simulink model "acf_force_control_simple"  (R2026b)
settings: Solver=ode4  StopTime=4  FixedStep=1.0000000000000001e-05
InitFcn:
  | acf_select_actuator(bdroot);
model workspace (MAT data in the model file):
  acfControlVersion = 'inertial-delivery-v8'
  acfImplementation = 'simple'
  acfLayoutVersion = 1
  p : object (value not decoded)
  pCompliant : object (value not decoded)
  pNearContact : object (value not decoded)
  pNoSprings : object (value not decoded)
  pRecommended : object (value not decoded)
symbols that are objects in the model workspace (value not decoded): p
undefined symbols (not defined in the file): DiscIntNeverNeededParam
(part 3 of 3)

== system acf_force_control_simple/Force controller/Coil PI and PID/Measured motion feedforward ==
  Acceleration FF audit native rate : ZeroOrderHold  SampleTime=p.sim.step
  Acceleration FF audit vector : Mux  Inputs=2
  Acceleration FF native log : ToWorkspace  VariableName=acceleration_feedforward_log  SaveFormat=Timeseries  SampleTime=-1
  Acceleration FF prediction time : Gain  Gain=p.inertial.accelerationPrediction_s
  Causal acceleration for current FF : Sum
  Filtered measured acceleration rate : DiscreteTransferFcn  Numerator=p.d.accelerationPrediction.derivativeNumerator  Denominator=p.d.accelerationPrediction.derivativeDenominator  SampleTime=p.force.sampleTime
  Geometry current feedforward : Gain  Gain=(p.contact.geometryFeedforwardScale/p.d.coilForceConstant_model_N_A)*double(p.force.feedforwardEnabled)
  Guide Coulomb friction current : Gain  Gain=(p.inertial.guideFrictionFeedforwardScale*p.coil.coulombForce/p.d.coilForceConstant_model_N_A)*double(p.force.feedforwardEnabled)
  Guide friction direction : Trigonometry  Operator=tanh
  Guide friction feedforward : Sum
  Guide friction velocity scale : Gain  Gain=1/p.coil.frictionSpeed
  Guide viscous friction current : Gain  Gain=(p.inertial.guideFrictionFeedforwardScale*p.coil.viscousFriction/p.d.coilForceConstant_model_N_A)*double(p.force.feedforwardEnabled)
  Identified guide prediction time : Gain  Gain=p.inertial.guideVelocityPrediction_s
  Measured acceleration current feedforward : Gain  Gain=(-p.inertial.accelerationFeedforwardScale*(p.d.identifiedHolderMass_kg+p.sensor.distalMass_model_kg)/p.d.coilForceConstant_model_N_A)*double(p.force.feedforwardEnabled)
  Measured head gap acceleration : Sum  Inputs=+-
  Predicted guide velocity : Sum
  acceleration_current_A : Outport
  geometry_current_A : Outport  Port=2
  friction_current_A : Outport  Port=3
  wires:
  Guide friction feedforward/1 -> friction_current_A/1
  Guide viscous friction current/1 -> Guide friction feedforward/1
  Acceleration FF audit native rate/1 -> Acceleration FF native log/1
  Guide friction direction/1 -> Guide Coulomb friction current/1
  Measured acceleration current feedforward/1 -> acceleration_current_A/1
  [inertial_robot_acceleration_aligned] -> Measured head gap acceleration/1
  [inertial_head_gap_velocity] -> Predicted guide velocity/1
  [measured_S_acceleration_z] -> Filtered measured acceleration rate/1, Acceleration FF audit vector/1, Measured head gap acceleration/2, Causal acceleration for current FF/1
  Geometry current feedforward/1 -> geometry_current_A/1
  Guide Coulomb friction current/1 -> Guide friction feedforward/2
  Measured head gap acceleration/1 -> Identified guide prediction time/1
  Filtered measured acceleration rate/1 -> Acceleration FF prediction time/1
  Guide friction velocity scale/1 -> Guide friction direction/1
  Identified guide prediction time/1 -> Predicted guide velocity/2
  Acceleration FF prediction time/1 -> Causal acceleration for current FF/2
  [inertial_axial_reference_deviation_N] -> Geometry current feedforward/1
  Acceleration FF audit vector/1 -> Acceleration FF audit native rate/1
  Predicted guide velocity/1 -> Guide friction velocity scale/1, Guide viscous friction current/1
  Causal acceleration for current FF/1 -> Acceleration FF audit vector/2, Measured acceleration current feedforward/1

== system acf_force_control_simple/Force controller/Coil PI and PID/Normal force PI and PID ==
  error_N : Inport
  anti_windup : Inport  Port=2
  Error to normal deviation : Gain  Gain=-1
  Normal error and anti windup : Sum
  Normal error derivative memory : UnitDelay  SampleTime=p.force.sampleTime
  Normal error filtered derivative : Sum
  Normal error new derivative weight : Gain  Gain=(1-exp(-p.force.sampleTime/p.inertial.derivativeFilter))/p.force.sampleTime
  Normal error old derivative weight : Gain  Gain=exp(-p.force.sampleTime/p.inertial.derivativeFilter)
  Normal error previous sample : UnitDelay  SampleTime=p.force.sampleTime
  Normal error sample increment : Sum  Inputs=+-
  Normal force derivative current : Gain  Gain=-p.inertial.forceKd*double(strcmp(p.coil.strategy,'pid'))
  Normal force error integral : DiscreteIntegrator  SampleTime=p.force.sampleTime  ICPrevOutput=DiscIntNeverNeededParam  ICPrevScaledInput=DiscIntNeverNeededParam
  Normal force integral current : Gain  Gain=-p.inertial.forceKi
  Normal force proportional current : Gain  Gain=-p.inertial.forceKp
  Optional feedback rolloff : DiscreteTransferFcn  Numerator=p.d.feedbackFilter.numerator  Denominator=p.d.feedbackFilter.denominator  InitialStates=p.d.feedbackFilter.initialStates  SampleTime=p.force.sampleTime
  PI and PID correction : Sum  Inputs=+++
  feedback_current_A : Outport
  wires:
  Optional feedback rolloff/1 -> feedback_current_A/1
  PI and PID correction/1 -> Optional feedback rolloff/1
  Normal force derivative current/1 -> PI and PID correction/3
  error_N/1 -> Error to normal deviation/1
  Normal error old derivative weight/1 -> Normal error filtered derivative/2
  anti_windup/1 -> Normal error and anti windup/2
  Normal error and anti windup/1 -> Normal force error integral/1
  Normal error derivative memory/1 -> Normal error old derivative weight/1
  Normal force proportional current/1 -> PI and PID correction/1
  Error to normal deviation/1 -> Normal force proportional current/1, Normal error previous sample/1, Normal error and anti windup/1, Normal error sample increment/1
  Normal error previous sample/1 -> Normal error sample increment/2
  Normal error filtered derivative/1 -> Normal error derivative memory/1, Normal force derivative current/1
  Normal force error integral/1 -> Normal force integral current/1
  Normal error sample increment/1 -> Normal error new derivative weight/1
  Normal force integral current/1 -> PI and PID correction/2
  Normal error new derivative weight/1 -> Normal error filtered derivative/1

== system acf_force_control_simple/Force controller/Screw normal PI and PID/Lower spring inverse feedforward ==
  Desired lower load deviation : Sum  Inputs=+-
  Full native inverse log : ToWorkspace  VariableName=lower_inverse_log  SaveFormat=Timeseries  SampleTime=-1
  Known downstream S inertia : Gain  Gain=p.sensor.distalMass_model_kg
  Native audit sampling : ZeroOrderHold  SampleTime=p.sim.step
  Native inverse audit : Mux
  Optional inverse feedforward scale : Gain  Gain=(double(p.inertial.lowerLoadInverse.enabled)*p.inertial.lowerLoadInverse.scale)*double(p.force.feedforwardEnabled)
  Proper identified lower-link inverse : DiscreteTransferFcn  Numerator=p.d.screwLowerLoadInverse.numerator  Denominator=p.d.screwLowerLoadInverse.denominator  InitialStates=zeros(3,1)  SampleTime=p.force.sampleTime
  extra_current_A : Outport
  wires:
  Native audit sampling/1 -> Full native inverse log/1
  Native inverse audit/1 -> Native audit sampling/1
  Optional inverse feedforward scale/1 -> extra_current_A/1, Native inverse audit/4
  Desired lower load deviation/1 -> Proper identified lower-link inverse/1, Native inverse audit/3
  [inertial_axial_reference_deviation_N] -> Desired lower load deviation/1, Native inverse audit/1
  Proper identified lower-link inverse/1 -> Optional inverse feedforward scale/1
  Known downstream S inertia/1 -> Desired lower load deviation/2, Native inverse audit/2
  [measured_S_acceleration_z] -> Known downstream S inertia/1

== system acf_force_control_simple/Force controller/Screw normal PI and PID/Measured motion feedforward ==
  Acceleration FF audit native rate : ZeroOrderHold  SampleTime=p.sim.step
  Acceleration FF audit vector : Mux  Inputs=2
  Acceleration FF native log : ToWorkspace  VariableName=acceleration_feedforward_log  SaveFormat=Timeseries  SampleTime=-1
  Acceleration FF prediction time : Gain  Gain=p.screw.accelerationPrediction_s
  Causal acceleration for current FF : Sum
  Combined measured acceleration current : Sum
  Filtered measured acceleration rate : DiscreteTransferFcn  Numerator=p.d.screwAccelerationPrediction.derivativeNumerator  Denominator=p.d.screwAccelerationPrediction.derivativeDenominator  SampleTime=p.force.sampleTime
  Geometry current feedforward : Gain  Gain=(p.contact.geometryFeedforwardScale/(p.d.screwTorqueConstant_model_Nm_A/p.d.ell))*double(p.force.feedforwardEnabled)
  Guide Coulomb friction current : Gain  Gain=(p.inertial.guideFrictionFeedforwardScale*(p.screw.coulombTorque/p.d.ell)/(p.d.screwTorqueConstant_model_Nm_A/p.d.ell))*double(p.force.feedforwardEnabled)
  Guide friction direction : Trigonometry  Operator=tanh
  Guide friction feedforward : Sum
  Guide friction velocity scale : Gain  Gain=1/(p.screw.frictionSpeed*p.d.ell)
  Guide viscous friction current : Gain  Gain=(p.inertial.guideFrictionFeedforwardScale*(p.screw.viscousTorque/p.d.ell^2)/(p.d.screwTorqueConstant_model_Nm_A/p.d.ell))*double(p.force.feedforwardEnabled)
  Identified guide prediction time : Gain  Gain=p.inertial.guideVelocityPrediction_s
  Measured acceleration current feedforward : Gain  Gain=(-p.inertial.accelerationFeedforwardScale*(p.d.identifiedHolderMass_kg+p.sensor.distalMass_model_kg+p.screw.rotorInertia/p.d.ell^2)*p.d.ell/p.d.screwTorqueConstant_model_Nm_A)*double(p.force.feedforwardEnabled)
  Measured head gap acceleration : Sum  Inputs=+-
  Predicted guide velocity : Sum
  Robot acceleration rotor current : Gain  Gain=(p.inertial.accelerationFeedforwardScale*p.screw.rotorInertia/(p.d.ell*p.d.screwTorqueConstant_model_Nm_A))*double(p.force.feedforwardEnabled)
  acceleration_current_A : Outport
  geometry_current_A : Outport  Port=2
  friction_current_A : Outport  Port=3
  wires:
  Guide Coulomb friction current/1 -> Guide friction feedforward/2
  Guide friction feedforward/1 -> friction_current_A/1
  Guide friction velocity scale/1 -> Guide friction direction/1
  [measured_S_acceleration_z] -> Filtered measured acceleration rate/1, Measured head gap acceleration/2, Acceleration FF audit vector/1, Causal acceleration for current FF/1
  Geometry current feedforward/1 -> geometry_current_A/1
  Guide viscous friction current/1 -> Guide friction feedforward/1
  [inertial_head_gap_velocity] -> Predicted guide velocity/1
  Causal acceleration for current FF/1 -> Acceleration FF audit vector/2, Measured acceleration current feedforward/1
  [inertial_robot_acceleration_aligned] -> Measured head gap acceleration/1, Robot acceleration rotor current/1
  Acceleration FF audit vector/1 -> Acceleration FF audit native rate/1
  Measured acceleration current feedforward/1 -> Combined measured acceleration current/2
  [inertial_axial_reference_deviation_N] -> Geometry current feedforward/1
  Filtered measured acceleration rate/1 -> Acceleration FF prediction time/1
  Acceleration FF audit native rate/1 -> Acceleration FF native log/1
  Measured head gap acceleration/1 -> Identified guide prediction time/1
  Combined measured acceleration current/1 -> acceleration_current_A/1
  Acceleration FF prediction time/1 -> Causal acceleration for current FF/2
  Identified guide prediction time/1 -> Predicted guide velocity/2
  Predicted guide velocity/1 -> Guide friction velocity scale/1, Guide viscous friction current/1
  Guide friction direction/1 -> Guide Coulomb friction current/1
  Robot acceleration rotor current/1 -> Combined measured acceleration current/1

== system acf_force_control_simple/Force controller/Screw normal PI and PID/Normal force PI and PID ==
  error_N : Inport
  anti_windup : Inport  Port=2
  Error to normal deviation : Gain  Gain=-1
  Feedback structural-mode filter : DiscreteTransferFcn  Numerator=p.d.screwFeedbackFilter.numerator  Denominator=p.d.screwFeedbackFilter.denominator  InitialStates=p.d.screwFeedbackFilter.initialStates  SampleTime=p.force.sampleTime
  Normal error and anti windup : Sum
  Normal error derivative memory : UnitDelay  SampleTime=p.force.sampleTime
  Normal error filtered derivative : Sum
  Normal error new derivative weight : Gain  Gain=(1-exp(-p.force.sampleTime/p.screw.currentDerivativeFilter))/p.force.sampleTime
  Normal error old derivative weight : Gain  Gain=exp(-p.force.sampleTime/p.screw.currentDerivativeFilter)
  Normal error previous sample : UnitDelay  SampleTime=p.force.sampleTime
  Normal error sample increment : Sum  Inputs=+-
  Normal force derivative current : Gain  Gain=-p.screw.currentForceKd*double(strcmp(p.coil.strategy,'pid'))
  Normal force error integral : DiscreteIntegrator  SampleTime=p.force.sampleTime  ICPrevOutput=DiscIntNeverNeededParam  ICPrevScaledInput=DiscIntNeverNeededParam
  Normal force integral current : Gain  Gain=-p.screw.currentForceKi
  Normal force proportional current : Gain  Gain=-p.screw.currentForceKp
  PI and PID correction : Sum  Inputs=+++
  feedback_current_A : Outport
  wires:
  Feedback structural-mode filter/1 -> feedback_current_A/1
  Normal error previous sample/1 -> Normal error sample increment/2
  Normal error and anti windup/1 -> Normal force error integral/1
  Normal error sample increment/1 -> Normal error new derivative weight/1
  Normal force integral current/1 -> PI and PID correction/2
  Normal force proportional current/1 -> PI and PID correction/1
  Normal force error integral/1 -> Normal force integral current/1
  Normal error filtered derivative/1 -> Normal force derivative current/1, Normal error derivative memory/1
  Normal error new derivative weight/1 -> Normal error filtered derivative/1
  error_N/1 -> Error to normal deviation/1
  Normal error old derivative weight/1 -> Normal error filtered derivative/2
  PI and PID correction/1 -> Feedback structural-mode filter/1
  Normal error derivative memory/1 -> Normal error old derivative weight/1
  Error to normal deviation/1 -> Normal error previous sample/1, Normal force proportional current/1, Normal error and anti windup/1, Normal error sample increment/1
  anti_windup/1 -> Normal error and anti windup/2
  Normal force derivative current/1 -> PI and PID correction/3

== system acf_force_control_simple/Recenter travel/Force settling gate/Fast force variation and dwell ==
  normal_error_N : Inport
  held_slow_stability : Inport  Port=2
  All force stability conditions : Logic  AllPortsSameDT=off  OutDataTypeStr=boolean
  Allowed force variance : Constant  Value=p.robot.forceGate.variation.rmsLimit_N^2
  Cap fast stable count : Saturate  UpperLimit=p.d.variationGate.dwellSamples  LowerLimit=0
  Fast continuous dwell completed : RelationalOperator  OutDataTypeStr=boolean  RndMeth=Simplest  InputSameDT=off
  Fast error sample : ZeroOrderHold  SampleTime=p.force.sampleTime
  Fast force variance : DiscreteTransferFcn  Numerator=p.d.variationGate.varianceNumerator  Denominator=p.d.variationGate.varianceDenominator  SampleTime=p.force.sampleTime
  Fast normal force mean : DiscreteTransferFcn  Numerator=p.d.variationGate.meanNumerator  Denominator=p.d.variationGate.meanDenominator  SampleTime=p.force.sampleTime
  Held slow stability at fast rate : ZeroOrderHold  SampleTime=p.force.sampleTime
  Normal force above target : Gain  Gain=-1
  Normal force deviation : Sum  Inputs=+-
  One more fast stable sample : Bias  Bias=1  SaturateOnIntegerOverflow=off
  Previous fast stable count : UnitDelay  SampleTime=p.force.sampleTime
  RMS force variation : Math  Operator=sqrt
  Required fast dwell count : Constant  Value=p.d.variationGate.dwellSamples
  Reset dwell at every fast instability : Switch  Threshold=.5  SaturateOnIntegerOverflow=off  InputSameDT=off
  Reset fast dwell : Constant  Value=0
  Squared normal force deviation : Math  Operator=square
  Variation acceptable : RelationalOperator  Operator=<=  OutDataTypeStr=boolean  RndMeth=Simplest  InputSameDT=off
  ready_fast : Outport
  mean_error_N : Outport  Port=2
  variation_rms_N : Outport  Port=3
  stable_sample_count : Outport  Port=4
  stable_fast : Outport  Port=5
  wires:
  One more fast stable sample/1 -> Reset dwell at every fast instability/1
  Previous fast stable count/1 -> One more fast stable sample/1
  Reset dwell at every fast instability/1 -> Cap fast stable count/1
  Reset fast dwell/1 -> Reset dwell at every fast instability/3
  Fast error sample/1 -> Normal force above target/1
  Allowed force variance/1 -> Variation acceptable/2
  All force stability conditions/1 -> stable_fast/1, Reset dwell at every fast instability/2
  Cap fast stable count/1 -> stable_sample_count/1, Fast continuous dwell completed/1, Previous fast stable count/1
  Fast normal force mean/1 -> mean_error_N/1, Normal force deviation/2
  Normal force deviation/1 -> Squared normal force deviation/1
  Squared normal force deviation/1 -> Fast force variance/1
  held_slow_stability/1 -> Held slow stability at fast rate/1
  Fast continuous dwell completed/1 -> ready_fast/1
  Required fast dwell count/1 -> Fast continuous dwell completed/2
  Fast force variance/1 -> Variation acceptable/1, RMS force variation/1
  RMS force variation/1 -> variation_rms_N/1
  normal_error_N/1 -> Fast error sample/1
  Normal force above target/1 -> Fast normal force mean/1, Normal force deviation/1
  Held slow stability at fast rate/1 -> All force stability conditions/1
  Variation acceptable/1 -> All force stability conditions/2
